simulink model "StarshipSystemModel"  (R2025b)
settings: Solver=VariableStepAuto  StartTime=0.0  StopTime=10.0  RelTol=1e-3
model workspace (MAT data in the model file):
  ActiveGNCMode : Simulink.Bus (value not decoded)
  AerodynamicControlCommand : Simulink.Bus (value not decoded)
  AerodynamicLoad : Simulink.Bus (value not decoded)
  AggregatedStream : Simulink.Bus (value not decoded)
  AllocatedEffectorDemand : Simulink.Bus (value not decoded)
  AttitudeControlDemand : Simulink.Bus (value not decoded)
  AttitudeGuidanceCommand : Simulink.Bus (value not decoded)
  AttitudeRateState : Simulink.Bus (value not decoded)
  AutogenousPressurantGas : Simulink.ConnectionBus (value not decoded)
  CandidateFaultIndication : Simulink.Bus (value not decoded)
  CombustionGasFeed : Simulink.ConnectionBus (value not decoded)
  CommandPathHealth : Simulink.Bus (value not decoded)
  ControlMode : Simulink.ValueType (value not decoded)
  DownlinkSignal : Simulink.Bus (value not decoded)
  ElectricalPower : Simulink.ConnectionBus (value not decoded)
  EngineTelemetry : Simulink.Bus (value not decoded)
  ExecutionContext : Simulink.Bus (value not decoded)
  FaultDiagnosisResult : Simulink.Bus (value not decoded)
  GNCDataContext : Simulink.Bus (value not decoded)
  GNCHealthState : Simulink.Bus (value not decoded)
  GNCStateEstimate : Simulink.Bus (value not decoded)
  GimbalAngle : Simulink.ValueType (value not decoded)
  GimbalMotion : Simulink.ConnectionBus (value not decoded)
  GroundCheckoutLink : Simulink.Bus (value not decoded)
  GroundPressurantSupply : Simulink.ConnectionBus (value not decoded)
  GuidanceConstraints : Simulink.Bus (value not decoded)
  GuidanceMode : Simulink.ValueType (value not decoded)
  LinkHealth : Simulink.Bus (value not decoded)
  LiquidPropellantFeed : Simulink.ConnectionBus (value not decoded)
  MechanicalMotion : Simulink.ConnectionBus (value not decoded)
  MechanismPosition : Simulink.Bus (value not decoded)
  ModeTransitionContext : Simulink.Bus (value not decoded)
  NavigationAidingData : Simulink.Bus (value not decoded)
  NavigationEstimate : Simulink.Bus (value not decoded)
  NavigationHealthStatus : Simulink.Bus (value not decoded)
  NavigationMeasurementSet : Simulink.Bus (value not decoded)
  PercentThrottle : Simulink.ValueType (value not decoded)
  PneumaticActuationGas : Simulink.ConnectionBus (value not decoded)
  PowerConversionStatus : Simulink.Bus (value not decoded)
  PowerDistributionStatus : Simulink.Bus (value not decoded)
  PowerHealthStatus : Simulink.Bus (value not decoded)
  PowerManagementCommand : Simulink.Bus (value not decoded)
  PowerStorageStatus : Simulink.Bus (value not decoded)
  ProtectedThermalState : Simulink.Bus (value not decoded)
  ProtectionIsolationStatus : Simulink.Bus (value not decoded)
  PurgeGasSupply : Simulink.ConnectionBus (value not decoded)
  RCSPulseCommand : Simulink.Bus (value not decoded)
  RCSTelemetry : Simulink.Bus (value not decoded)
  RFFeed : Simulink.ConnectionBus (value not decoded)
  RecoveryMechanismCommand : Simulink.Bus (value not decoded)
  RollThrottleBias : Simulink.ValueType (value not decoded)
  SafetyOverride : Simulink.ValueType (value not decoded)
  SafetyStateStatus : Simulink.Bus (value not decoded)
  ShapedControlDemand : Simulink.Bus (value not decoded)
  SpinStartIgniterGas : Simulink.ConnectionBus (value not decoded)
  StageMechanicalBoundary : Simulink.ConnectionBus (value not decoded)
  StructuralLoad : Simulink.ConnectionBus (value not decoded)
  StructureHealthStatus : Simulink.Bus (value not decoded)
  SubsystemHealthEvidence : Simulink.Bus (value not decoded)
  SubsystemStatusTelemetry : Simulink.Bus (value not decoded)
  TankTelemetry : Simulink.Bus (value not decoded)
  ThermalMonitoringCommand : Simulink.Bus (value not decoded)
  ThermalNetwork : Simulink.ConnectionBus (value not decoded)
  ThrustLoad : Simulink.ConnectionBus (value not decoded)
  TrajectoryGuidanceCommand : Simulink.Bus (value not decoded)
  TrajectoryReference : Simulink.Bus (value not decoded)
  TranslationalControlDemand : Simulink.Bus (value not decoded)
  TranslationalState : Simulink.Bus (value not decoded)
  UplinkSignal : Simulink.Bus (value not decoded)
  ValidatedControlDemand : Simulink.Bus (value not decoded)
  ValveCommand : Simulink.ValueType (value not decoded)
  VehicleStructureState : Simulink.Bus (value not decoded)
  VerifiedCommand : Simulink.Bus (value not decoded)
  VideoStream : Simulink.Bus (value not decoded)
undefined symbols (not defined in the file): ACR, ACT, ASM, ATM, BCR, BDQ, BDR, BDX, BEC, BFC, BHV, BIP, BLM, BNZ, BPI, BPR, BPV, BRX, BSM, BTA, BTP, BVC, BVE, BVV, CAA, CAM, CAS, CAT, CLM, COM, CRS, CTL, CTR, DAQ, ESC, EXT, FCR, FDB, FDE, FEX, FHI, FHM, FIC, FIS, FMG, FSC, GAP, GCM, GMD, GNC, GND, GPH, GTR, HDN, HIA, HSI, IF, INT, LOC, NAI ... (+45)
(part 3 of 8)

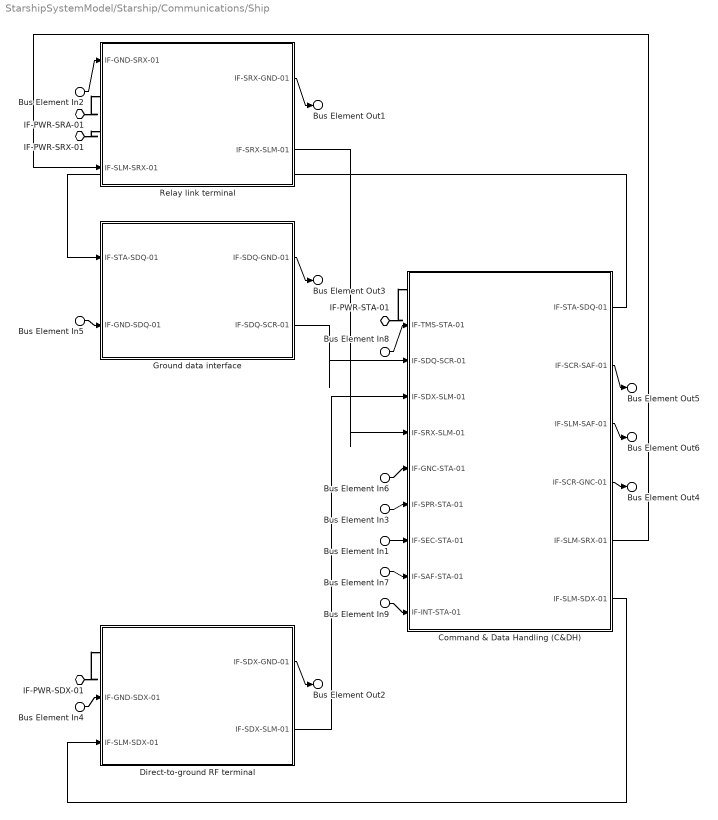
== system StarshipSystemModel/Starship/Communications/Ship ==
  Bus Element In8 : Inport  PortName=IF-TMS-STA-01
  Bus Element In6 : Inport  Port=2  PortName=IF-GNC-STA-01
  Bus Element In3 : Inport  Port=3  PortName=IF-SPR-STA-01
  Bus Element In1 : Inport  Port=4  PortName=IF-SEC-STA-01
  Bus Element In2 : Inport  Port=5  PortName=IF-GND-SRX-01
  Bus Element In4 : Inport  Port=6  PortName=IF-GND-SDX-01
  Bus Element In5 : Inport  Port=7  PortName=IF-GND-SDQ-01
  Bus Element In7 : Inport  Port=8  PortName=IF-SAF-STA-01
  Bus Element In9 : Inport  Port=9  PortName=IF-INT-STA-01
  Command & Data Handling (C&DH) : Subsystem
      settings: PortSchema="{\"entries\":[{\"content\":{\"headerSize\":26,\"margin\":15,\"minimumSpacing\":25,\"sides\":[{\"content\":{\"connectorIds\":[\"LConn1\",\"In1\",\"In2\",\"In3\",\"In4\",\"In5\",\"In6\",\"In7\",\"In8\",\"In9\"]},\"type\":\"ConnectorPlacement.EquallySpacedRectSide\",\"uuid\":\"57d8a002-ec9a-4125-b797-7e7c6712bf02\"},{\"content\":{\"connectorIds\":[\"Out1\",\"Out2\",\"Out3\",\"Out4\",\"Out5\",\"Out6\"],\"side\":\"RIGHT\"},\"type\":\"ConnectorPlacement.EquallySpacedRectSide\",\"uuid\":\"9c166a96-12fc-4382-8ebe-da88da7fda26\"},{\"content\":{\"side\":\"TOP\"},\"type\":\"ConnectorPlacement.EquallySpacedRectSide\",\"uuid\":\"d709cb41-f5aa-4a2a-ad2b-35894222a9c1\"}]},\"type\":\"ConnectorPlacement.EquallySpacedConnector\",\"uuid\":\"04bb3772-118b-42d1-ac15-43c1b901053a\"}],\"packageUris\":[\"http://schema.mathworks.com/mf0/Connector/R2020b\"],\"version\":\"1.0\"}"
  Direct-to-ground RF terminal : Subsystem
      settings: PortSchema="{\"entries\":[{\"content\":{\"headerSize\":26,\"margin\":15,\"minimumSpacing\":25,\"sides\":[{\"content\":{\"connectorIds\":[\"LConn1\",\"In1\",\"In2\"]},\"type\":\"ConnectorPlacement.EquallySpacedRectSide\",\"uuid\":\"57d8a002-ec9a-4125-b797-7e7c6712bf02\"},{\"content\":{\"connectorIds\":[\"Out1\",\"Out2\"],\"side\":\"RIGHT\"},\"type\":\"ConnectorPlacement.EquallySpacedRectSide\",\"uuid\":\"9c166a96-12fc-4382-8ebe-da88da7fda26\"},{\"content\":{\"side\":\"TOP\"},\"type\":\"ConnectorPlacement.EquallySpacedRectSide\",\"uuid\":\"d709cb41-f5aa-4a2a-ad2b-35894222a9c1\"}]},\"type\":\"ConnectorPlacement.EquallySpacedConnector\",\"uuid\":\"04bb3772-118b-42d1-ac15-43c1b901053a\"}],\"packageUris\":[\"http://schema.mathworks.com/mf0/Connector/R2020b\"],\"version\":\"1.0\"}"
  Ground data interface : Subsystem
      settings: PortSchema="{\"entries\":[{\"content\":{\"headerSize\":26,\"margin\":15,\"minimumSpacing\":25,\"sides\":[{\"content\":{\"connectorIds\":[\"In1\",\"In2\"]},\"type\":\"ConnectorPlacement.EquallySpacedRectSide\",\"uuid\":\"57d8a002-ec9a-4125-b797-7e7c6712bf02\"},{\"content\":{\"connectorIds\":[\"Out1\",\"Out2\"],\"side\":\"RIGHT\"},\"type\":\"ConnectorPlacement.EquallySpacedRectSide\",\"uuid\":\"9c166a96-12fc-4382-8ebe-da88da7fda26\"},{\"content\":{\"side\":\"TOP\"},\"type\":\"ConnectorPlacement.EquallySpacedRectSide\",\"uuid\":\"d709cb41-f5aa-4a2a-ad2b-35894222a9c1\"}]},\"type\":\"ConnectorPlacement.EquallySpacedConnector\",\"uuid\":\"04bb3772-118b-42d1-ac15-43c1b901053a\"}],\"packageUris\":[\"http://schema.mathworks.com/mf0/Connector/R2020b\"],\"version\":\"1.0\"}"
  Relay link terminal : Subsystem
      settings: PortSchema="{\"entries\":[{\"content\":{\"headerSize\":26,\"margin\":15,\"minimumSpacing\":25,\"sides\":[{\"content\":{\"connectorIds\":[\"In1\",\"LConn1\",\"LConn2\",\"In2\"]},\"type\":\"ConnectorPlacement.EquallySpacedRectSide\",\"uuid\":\"57d8a002-ec9a-4125-b797-7e7c6712bf02\"},{\"content\":{\"connectorIds\":[\"Out1\",\"Out2\"],\"side\":\"RIGHT\"},\"type\":\"ConnectorPlacement.EquallySpacedRectSide\",\"uuid\":\"9c166a96-12fc-4382-8ebe-da88da7fda26\"},{\"content\":{\"side\":\"TOP\"},\"type\":\"ConnectorPlacement.EquallySpacedRectSide\",\"uuid\":\"d709cb41-f5aa-4a2a-ad2b-35894222a9c1\"}]},\"type\":\"ConnectorPlacement.EquallySpacedConnector\",\"uuid\":\"04bb3772-118b-42d1-ac15-43c1b901053a\"}],\"packageUris\":[\"http://schema.mathworks.com/mf0/Connector/R2020b\"],\"version\":\"1.0\"}"
  IF-PWR-SRA-01 : PMIOPort  Side=Left  ConnectionType=Bus: ElectricalPower
  IF-PWR-SRX-01 : PMIOPort  Port=2  Side=Left  ConnectionType=Bus: ElectricalPower
  IF-PWR-SDX-01 : PMIOPort  Port=3  Side=Left  ConnectionType=Bus: ElectricalPower
  IF-PWR-STA-01 : PMIOPort  Port=4  Side=Left  ConnectionType=Bus: ElectricalPower
  Bus Element Out2 : Outport  PortName=IF-SDX-GND-01
  Bus Element Out1 : Outport  Port=2  PortName=IF-SRX-GND-01
  Bus Element Out3 : Outport  Port=3  PortName=IF-SDQ-GND-01
  Bus Element Out4 : Outport  Port=4  PortName=IF-SCR-GNC-01
  Bus Element Out5 : Outport  Port=5  PortName=IF-SCR-SAF-01
  Bus Element Out6 : Outport  Port=6  PortName=IF-SLM-SAF-01
  wires:
  Relay link terminal/2(IF-SRX-SLM-01) -> Command & Data Handling (C&DH)/4(IF-SRX-SLM-01)
  Bus Element In1/1 -> Command & Data Handling (C&DH)/7(IF-SEC-STA-01)
  Relay link terminal/1(IF-SRX-GND-01) -> Bus Element Out1/1
  Bus Element In2/1 -> Relay link terminal/1(IF-GND-SRX-01)
  Command & Data Handling (C&DH)/4(IF-SCR-GNC-01) -> Bus Element Out4/1
  Bus Element In5/1 -> Ground data interface/2(IF-GND-SDQ-01)
  Command & Data Handling (C&DH)/2(IF-SCR-SAF-01) -> Bus Element Out5/1
  Bus Element In4/1 -> Direct-to-ground RF terminal/1(IF-GND-SDX-01)
  Ground data interface/1(IF-SDQ-GND-01) -> Bus Element Out3/1
  Ground data interface/2(IF-SDQ-SCR-01) -> Command & Data Handling (C&DH)/2(IF-SDQ-SCR-01)
  Bus Element In6/1 -> Command & Data Handling (C&DH)/5(IF-GNC-STA-01)
  Bus Element In3/1 -> Command & Data Handling (C&DH)/6(IF-SPR-STA-01)
  Command & Data Handling (C&DH)/6(IF-SLM-SDX-01) -> Direct-to-ground RF terminal/2(IF-SLM-SDX-01)
  Bus Element In7/1 -> Command & Data Handling (C&DH)/8(IF-SAF-STA-01)
  Direct-to-ground RF terminal/1(IF-SDX-GND-01) -> Bus Element Out2/1
  Direct-to-ground RF terminal/2(IF-SDX-SLM-01) -> Command & Data Handling (C&DH)/3(IF-SDX-SLM-01)
  Command & Data Handling (C&DH)/1(IF-STA-SDQ-01) -> Ground data interface/1(IF-STA-SDQ-01)
  Command & Data Handling (C&DH)/3(IF-SLM-SAF-01) -> Bus Element Out6/1
  Command & Data Handling (C&DH)/5(IF-SLM-SRX-01) -> Relay link terminal/2(IF-SLM-SRX-01)
  Bus Element In8/1 -> Command & Data Handling (C&DH)/1(IF-TMS-STA-01)
  Bus Element In9/1 -> Command & Data Handling (C&DH)/9(IF-INT-STA-01)
  connections:
  IF-PWR-SRA-01/RConn1 -- Relay link terminal/LConn1
  IF-PWR-SRX-01/RConn1 -- Relay link terminal/LConn2
  IF-PWR-SDX-01/RConn1 -- Direct-to-ground RF terminal/LConn1
  IF-PWR-STA-01/RConn1 -- Command & Data Handling (C&DH)/LConn1

== system StarshipSystemModel/Starship/GNC/Control Command & Allocation ==
  Bus Element In1 : Inport  PortName=IF-CLM-CAS-01
  Actuator / Subsystem Command Routing : Subsystem
      settings: PortSchema="{\"entries\":[{\"content\":{\"headerSize\":26,\"margin\":15,\"minimumSpacing\":25,\"sides\":[{\"content\":{\"connectorIds\":[\"In1\",\"LConn1\"]},\"type\":\"ConnectorPlacement.EquallySpacedRectSide\",\"uuid\":\"bfc9b5ca-65d3-4883-965c-09cadc06ae86\"},{\"content\":{\"connectorIds\":[\"Out1\",\"Out2\",\"Out3\",\"Out4\",\"Out5\",\"Out6\",\"Out7\",\"Out8\",\"Out9\",\"Out10\"],\"side\":\"RIGHT\"},\"type\":\"ConnectorPlacement.EquallySpacedRectSide\",\"uuid\":\"302eddba-73e5-4bab-ba05-7a4cd66d036f\"},{\"content\":{\"side\":\"TOP\"},\"type\":\"ConnectorPlacement.EquallySpacedRectSide\",\"uuid\":\"ad98d540-1dfa-45ea-9ded-5f35e32eb634\"}]},\"type\":\"ConnectorPlacement.EquallySpacedConnector\",\"uuid\":\"1bda90bf-7ec8-4676-b4c1-6df6810f307f\"}],\"packageUris\":[\"http://schema.mathworks.com/mf0/Connector/R2020b\"],\"version\":\"1.0\"}"
  Command Shaping & Limiting : Subsystem
      settings: PortSchema="{\"entries\":[{\"content\":{\"headerSize\":26,\"margin\":15,\"minimumSpacing\":25,\"sides\":[{\"content\":{\"connectorIds\":[\"In1\"]},\"type\":\"ConnectorPlacement.EquallySpacedRectSide\",\"uuid\":\"bfc9b5ca-65d3-4883-965c-09cadc06ae86\"},{\"content\":{\"connectorIds\":[\"Out1\"],\"side\":\"RIGHT\"},\"type\":\"ConnectorPlacement.EquallySpacedRectSide\",\"uuid\":\"302eddba-73e5-4bab-ba05-7a4cd66d036f\"},{\"content\":{\"side\":\"TOP\"},\"type\":\"ConnectorPlacement.EquallySpacedRectSide\",\"uuid\":\"ad98d540-1dfa-45ea-9ded-5f35e32eb634\"}]},\"type\":\"ConnectorPlacement.EquallySpacedConnector\",\"uuid\":\"1bda90bf-7ec8-4676-b4c1-6df6810f307f\"}],\"packageUris\":[\"http://schema.mathworks.com/mf0/Connector/R2020b\"],\"version\":\"1.0\"}"
  Control Allocation : Subsystem
      settings: PortSchema="{\"entries\":[{\"content\":{\"headerSize\":26,\"margin\":15,\"minimumSpacing\":25,\"sides\":[{\"content\":{\"connectorIds\":[\"In1\"]},\"type\":\"ConnectorPlacement.EquallySpacedRectSide\",\"uuid\":\"bfc9b5ca-65d3-4883-965c-09cadc06ae86\"},{\"content\":{\"connectorIds\":[\"Out1\"],\"side\":\"RIGHT\"},\"type\":\"ConnectorPlacement.EquallySpacedRectSide\",\"uuid\":\"302eddba-73e5-4bab-ba05-7a4cd66d036f\"},{\"content\":{\"side\":\"TOP\"},\"type\":\"ConnectorPlacement.EquallySpacedRectSide\",\"uuid\":\"ad98d540-1dfa-45ea-9ded-5f35e32eb634\"}]},\"type\":\"ConnectorPlacement.EquallySpacedConnector\",\"uuid\":\"1bda90bf-7ec8-4676-b4c1-6df6810f307f\"}],\"packageUris\":[\"http://schema.mathworks.com/mf0/Connector/R2020b\"],\"version\":\"1.0\"}"
  IF-PWR-GNC-01 : PMIOPort  Side=Left  ConnectionType=Bus: ElectricalPower
  Bus Element Out9 : Outport  PortName=IF-GNC-SPR-01
  Bus Element Out8 : Outport  Port=2  PortName=IF-GNC-BPR-01
  Bus Element Out7 : Outport  Port=3  PortName=IF-GNC-SFC-01
  Bus Element Out6 : Outport  Port=4  PortName=IF-GNC-BFC-01
  Bus Element Out5 : Outport  Port=5  PortName=IF-GNC-RCT-01
  Bus Element Out4 : Outport  Port=6  PortName=IF-GNC-TVC-01
  Bus Element Out3 : Outport  Port=7  PortName=IF-GNC-SEC-01
  Bus Element Out2 : Outport  Port=8  PortName=IF-GNC-BEC-01
  Bus Element Out1 : Outport  Port=9  PortName=IF-CRS-FHM-01
  Bus Element Out10 : Outport  Port=10  PortName=IF-GNC-ACT-01
  wires:
  Actuator / Subsystem Command Routing/4(IF-GNC-BFC-01) -> Bus Element Out6/1
  Actuator / Subsystem Command Routing/2(IF-GNC-BPR-01) -> Bus Element Out8/1
  Command Shaping & Limiting/1(IF-CAS-CAA-01) -> Control Allocation/1(IF-CAS-CAA-01)
  Bus Element In1/1 -> Command Shaping & Limiting/1(IF-CLM-CAS-01)
  Actuator / Subsystem Command Routing/5(IF-GNC-RCT-01) -> Bus Element Out5/1
  Actuator / Subsystem Command Routing/3(IF-GNC-SFC-01) -> Bus Element Out7/1
  Actuator / Subsystem Command Routing/1(IF-GNC-SPR-01) -> Bus Element Out9/1
  Actuator / Subsystem Command Routing/7(IF-GNC-SEC-01) -> Bus Element Out3/1
  Control Allocation/1(IF-CAA-CRS-01) -> Actuator / Subsystem Command Routing/1(IF-CAA-CRS-01)
  Actuator / Subsystem Command Routing/6(IF-GNC-TVC-01) -> Bus Element Out4/1
  Actuator / Subsystem Command Routing/8(IF-GNC-BEC-01) -> Bus Element Out2/1
  Actuator / Subsystem Command Routing/9(IF-CRS-FHM-01) -> Bus Element Out1/1
  Actuator / Subsystem Command Routing/10(IF-GNC-ACT-01) -> Bus Element Out10/1
  connections:
  IF-PWR-GNC-01/RConn1 -- Actuator / Subsystem Command Routing/LConn1

== system StarshipSystemModel/Starship/GNC/Flight Control ==
  Bus Element In3 : Inport  PortName=IF-GPH-CAT-01
  Bus Element In4 : Inport  Port=2  PortName=IF-GPH-CTR-01
  Bus Element In2 : Inport  Port=3  PortName=IF-NSE-CTR-01
  Bus Element In1 : Inport  Port=4  PortName=IF-NSE-CAT-01
  Bus Element In5 : Inport  Port=5  PortName=IF-FMG-CAM-01
  Attitude / Rate Control : Subsystem
      settings: PortSchema="{\"entries\":[{\"content\":{\"headerSize\":26,\"margin\":15,\"minimumSpacing\":25,\"sides\":[{\"content\":{\"connectorIds\":[\"In1\",\"In2\",\"In3\"]},\"type\":\"ConnectorPlacement.EquallySpacedRectSide\",\"uuid\":\"bfc9b5ca-65d3-4883-965c-09cadc06ae86\"},{\"content\":{\"connectorIds\":[\"Out1\"],\"side\":\"RIGHT\"},\"type\":\"ConnectorPlacement.EquallySpacedRectSide\",\"uuid\":\"302eddba-73e5-4bab-ba05-7a4cd66d036f\"},{\"content\":{\"side\":\"TOP\"},\"type\":\"ConnectorPlacement.EquallySpacedRectSide\",\"uuid\":\"ad98d540-1dfa-45ea-9ded-5f35e32eb634\"}]},\"type\":\"ConnectorPlacement.EquallySpacedConnector\",\"uuid\":\"1bda90bf-7ec8-4676-b4c1-6df6810f307f\"}],\"packageUris\":[\"http://schema.mathworks.com/mf0/Connector/R2020b\"],\"version\":\"1.0\"}"
  Control-Law Monitoring & Limiting : Subsystem
      settings: PortSchema="{\"entries\":[{\"content\":{\"headerSize\":26,\"margin\":15,\"minimumSpacing\":25,\"sides\":[{\"content\":{\"connectorIds\":[\"In1\",\"In2\"]},\"type\":\"ConnectorPlacement.EquallySpacedRectSide\",\"uuid\":\"bfc9b5ca-65d3-4883-965c-09cadc06ae86\"},{\"content\":{\"connectorIds\":[\"Out1\"],\"side\":\"RIGHT\"},\"type\":\"ConnectorPlacement.EquallySpacedRectSide\",\"uuid\":\"302eddba-73e5-4bab-ba05-7a4cd66d036f\"},{\"content\":{\"side\":\"TOP\"},\"type\":\"ConnectorPlacement.EquallySpacedRectSide\",\"uuid\":\"ad98d540-1dfa-45ea-9ded-5f35e32eb634\"}]},\"type\":\"ConnectorPlacement.EquallySpacedConnector\",\"uuid\":\"1bda90bf-7ec8-4676-b4c1-6df6810f307f\"}],\"packageUris\":[\"http://schema.mathworks.com/mf0/Connector/R2020b\"],\"version\":\"1.0\"}"
  Control-Mode Management : Subsystem
      settings: PortSchema="{\"entries\":[{\"content\":{\"headerSize\":26,\"margin\":15,\"minimumSpacing\":25,\"sides\":[{\"content\":{\"connectorIds\":[\"In1\"]},\"type\":\"ConnectorPlacement.EquallySpacedRectSide\",\"uuid\":\"bfc9b5ca-65d3-4883-965c-09cadc06ae86\"},{\"content\":{\"connectorIds\":[\"Out1\",\"Out2\"],\"side\":\"RIGHT\"},\"type\":\"ConnectorPlacement.EquallySpacedRectSide\",\"uuid\":\"302eddba-73e5-4bab-ba05-7a4cd66d036f\"},{\"content\":{\"side\":\"TOP\"},\"type\":\"ConnectorPlacement.EquallySpacedRectSide\",\"uuid\":\"ad98d540-1dfa-45ea-9ded-5f35e32eb634\"}]},\"type\":\"ConnectorPlacement.EquallySpacedConnector\",\"uuid\":\"1bda90bf-7ec8-4676-b4c1-6df6810f307f\"}],\"packageUris\":[\"http://schema.mathworks.com/mf0/Connector/R2020b\"],\"version\":\"1.0\"}"
  Trajectory / Translational Control : Subsystem
      settings: PortSchema="{\"entries\":[{\"content\":{\"headerSize\":26,\"margin\":15,\"minimumSpacing\":25,\"sides\":[{\"content\":{\"connectorIds\":[\"In1\",\"In2\",\"In3\"]},\"type\":\"ConnectorPlacement.EquallySpacedRectSide\",\"uuid\":\"bfc9b5ca-65d3-4883-965c-09cadc06ae86\"},{\"content\":{\"connectorIds\":[\"Out1\"],\"side\":\"RIGHT\"},\"type\":\"ConnectorPlacement.EquallySpacedRectSide\",\"uuid\":\"302eddba-73e5-4bab-ba05-7a4cd66d036f\"},{\"content\":{\"side\":\"TOP\"},\"type\":\"ConnectorPlacement.EquallySpacedRectSide\",\"uuid\":\"ad98d540-1dfa-45ea-9ded-5f35e32eb634\"}]},\"type\":\"ConnectorPlacement.EquallySpacedConnector\",\"uuid\":\"1bda90bf-7ec8-4676-b4c1-6df6810f307f\"}],\"packageUris\":[\"http://schema.mathworks.com/mf0/Connector/R2020b\"],\"version\":\"1.0\"}"
  Bus Element Out1 : Outport  PortName=IF-CLM-CAS-01
  wires:
  Bus Element In1/1 -> Attitude / Rate Control/2(IF-NSE-CAT-01)
  Bus Element In4/1 -> Trajectory / Translational Control/2(IF-GPH-CTR-01)
  Control-Mode Management/1(IF-CAM-CAT-01) -> Attitude / Rate Control/3(IF-CAM-CAT-01)
  Bus Element In3/1 -> Attitude / Rate Control/1(IF-GPH-CAT-01)
  Bus Element In2/1 -> Trajectory / Translational Control/1(IF-NSE-CTR-01)
  Bus Element In5/1 -> Control-Mode Management/1(IF-FMG-CAM-01)
  Control-Mode Management/2(IF-CAM-CTR-01) -> Trajectory / Translational Control/3(IF-CAM-CTR-01)
  Trajectory / Translational Control/1(IF-CTR-CLM-01) -> Control-Law Monitoring & Limiting/1(IF-CTR-CLM-01)
  Attitude / Rate Control/1(IF-CAT-CLM-01) -> Control-Law Monitoring & Limiting/2(IF-CAT-CLM-01)
  Control-Law Monitoring & Limiting/1(IF-CLM-CAS-01) -> Bus Element Out1/1

== system StarshipSystemModel/Starship/GNC/GNC Flight Software & Mode Management ==
  Bus Element In6 : Inport  PortName=IF-SAF-FHM-01
  Bus Element In5 : Inport  Port=2  PortName=IF-SCR-GNC-01
  Bus Element In4 : Inport  Port=3  PortName=IF-BCR-GNC-01
  Bus Element In3 : Inport  Port=4  PortName=IF-TVC-GNC-01
  Bus Element In1 : Inport  Port=5  PortName=IF-NVI-FHM-01
  Bus Element In2 : Inport  Port=6  PortName=IF-CRS-FHM-01
  GNC Data & Interface Management : Subsystem
      settings: PortSchema="{\"entries\":[{\"content\":{\"headerSize\":26,\"margin\":15,\"minimumSpacing\":25,\"sides\":[{\"content\":{\"connectorIds\":[\"In2\",\"In1\",\"In3\"]},\"type\":\"ConnectorPlacement.EquallySpacedRectSide\",\"uuid\":\"bfc9b5ca-65d3-4883-965c-09cadc06ae86\"},{\"content\":{\"connectorIds\":[\"Out1\",\"Out2\",\"Out3\"],\"side\":\"RIGHT\"},\"type\":\"ConnectorPlacement.EquallySpacedRectSide\",\"uuid\":\"302eddba-73e5-4bab-ba05-7a4cd66d036f\"},{\"content\":{\"side\":\"TOP\"},\"type\":\"ConnectorPlacement.EquallySpacedRectSide\",\"uuid\":\"ad98d540-1dfa-45ea-9ded-5f35e32eb634\"},{\"content\":{\"side\":\"BOTTOM\"},\"type\":\"ConnectorPlacement.EquallySpacedRectSide\",\"uuid\":\"ee596e90-1eb5-469d-9fa4-539f9d2bb748\"}]},\"type\":\"ConnectorPlacement.EquallySpacedConnector\",\"uuid\":\"1bda90bf-7ec8-4676-b4c1-6df6810f307f\"}],\"packageUris\":[\"http://schema.mathworks.com/mf0/Connector/R2020b\"],\"version\":\"1.0\"}"
  GNC Function Execution : Subsystem
      settings: PortSchema="{\"entries\":[{\"content\":{\"headerSize\":26,\"margin\":15,\"minimumSpacing\":25,\"sides\":[{\"content\":{\"connectorIds\":[\"In1\"]},\"type\":\"ConnectorPlacement.EquallySpacedRectSide\",\"uuid\":\"bfc9b5ca-65d3-4883-965c-09cadc06ae86\"},{\"content\":{\"connectorIds\":[\"Out1\"],\"side\":\"RIGHT\"},\"type\":\"ConnectorPlacement.EquallySpacedRectSide\",\"uuid\":\"302eddba-73e5-4bab-ba05-7a4cd66d036f\"},{\"content\":{\"side\":\"TOP\"},\"type\":\"ConnectorPlacement.EquallySpacedRectSide\",\"uuid\":\"ad98d540-1dfa-45ea-9ded-5f35e32eb634\"}]},\"type\":\"ConnectorPlacement.EquallySpacedConnector\",\"uuid\":\"1bda90bf-7ec8-4676-b4c1-6df6810f307f\"}],\"packageUris\":[\"http://schema.mathworks.com/mf0/Connector/R2020b\"],\"version\":\"1.0\"}"
  GNC Health Monitoring / Fault Response : Subsystem
      settings: PortSchema="{\"entries\":[{\"content\":{\"headerSize\":26,\"margin\":15,\"minimumSpacing\":25,\"sides\":[{\"content\":{\"connectorIds\":[\"In1\",\"In2\",\"In3\"]},\"type\":\"ConnectorPlacement.EquallySpacedRectSide\",\"uuid\":\"bfc9b5ca-65d3-4883-965c-09cadc06ae86\"},{\"content\":{\"connectorIds\":[\"Out1\",\"Out2\",\"Out3\"],\"side\":\"RIGHT\"},\"type\":\"ConnectorPlacement.EquallySpacedRectSide\",\"uuid\":\"302eddba-73e5-4bab-ba05-7a4cd66d036f\"},{\"content\":{\"side\":\"TOP\"},\"type\":\"ConnectorPlacement.EquallySpacedRectSide\",\"uuid\":\"ad98d540-1dfa-45ea-9ded-5f35e32eb634\"}]},\"type\":\"ConnectorPlacement.EquallySpacedConnector\",\"uuid\":\"1bda90bf-7ec8-4676-b4c1-6df6810f307f\"}],\"packageUris\":[\"http://schema.mathworks.com/mf0/Connector/R2020b\"],\"version\":\"1.0\"}"
  GNC Mode Management : Subsystem
      settings: PortSchema="{\"entries\":[{\"content\":{\"headerSize\":26,\"margin\":15,\"minimumSpacing\":25,\"sides\":[{\"content\":{\"connectorIds\":[\"In1\",\"In2\"]},\"type\":\"ConnectorPlacement.EquallySpacedRectSide\",\"uuid\":\"bfc9b5ca-65d3-4883-965c-09cadc06ae86\"},{\"content\":{\"connectorIds\":[\"Out1\",\"Out2\"],\"side\":\"RIGHT\"},\"type\":\"ConnectorPlacement.EquallySpacedRectSide\",\"uuid\":\"302eddba-73e5-4bab-ba05-7a4cd66d036f\"},{\"content\":{\"side\":\"TOP\"},\"type\":\"ConnectorPlacement.EquallySpacedRectSide\",\"uuid\":\"ad98d540-1dfa-45ea-9ded-5f35e32eb634\"}]},\"type\":\"ConnectorPlacement.EquallySpacedConnector\",\"uuid\":\"1bda90bf-7ec8-4676-b4c1-6df6810f307f\"}],\"packageUris\":[\"http://schema.mathworks.com/mf0/Connector/R2020b\"],\"version\":\"1.0\"}"
  Bus Element Out5 : Outport  PortName=IF-GNC-TMS-01
  Bus Element Out4 : Outport  Port=2  PortName=IF-GNC-STA-01
  Bus Element Out3 : Outport  Port=3  PortName=IF-GNC-BTA-01
  Bus Element Out1 : Outport  Port=4  PortName=IF-FMG-GMD-01
  Bus Element Out2 : Outport  Port=5  PortName=IF-FMG-CAM-01
  Bus Element Out6 : Outport  Port=6  PortName=IF-FHM-SAF-01
  wires:
  GNC Health Monitoring / Fault Response/2(IF-GNC-TMS-01) -> Bus Element Out5/1
  Bus Element In2/1 -> GNC Health Monitoring / Fault Response/3(IF-CRS-FHM-01)
  Bus Element In1/1 -> GNC Health Monitoring / Fault Response/2(IF-NVI-FHM-01)
  GNC Data & Interface Management/3(IF-GNC-STA-01) -> Bus Element Out4/1
  GNC Data & Interface Management/1(IF-FDB-FEX-01) -> GNC Function Execution/1(IF-FDB-FEX-01)
  GNC Health Monitoring / Fault Response/1(IF-FHM-FMG-01) -> GNC Mode Management/2(IF-FHM-FMG-01)
  GNC Function Execution/1(IF-FEX-FMG-01) -> GNC Mode Management/1(IF-FEX-FMG-01)
  GNC Data & Interface Management/2(IF-GNC-BTA-01) -> Bus Element Out3/1
  GNC Mode Management/1(IF-FMG-GMD-01) -> Bus Element Out1/1
  GNC Mode Management/2(IF-FMG-CAM-01) -> Bus Element Out2/1
  Bus Element In5/1 -> GNC Data & Interface Management/2(IF-SCR-GNC-01)
  Bus Element In4/1 -> GNC Data & Interface Management/1(IF-BCR-GNC-01)
  Bus Element In3/1 -> GNC Data & Interface Management/3(IF-TVC-GNC-01)
  GNC Health Monitoring / Fault Response/3(IF-FHM-SAF-01) -> Bus Element Out6/1
  Bus Element In6/1 -> GNC Health Monitoring / Fault Response/1(IF-SAF-FHM-01)

== system StarshipSystemModel/Starship/GNC/Guidance & Trajectory Management ==
  Bus Element In1 : Inport  PortName=IF-NSE-GPH-01
  Bus Element In2 : Inport  Port=2  PortName=IF-FMG-GMD-01
  Flight-Phase Guidance : Subsystem
      settings: PortSchema="{\"entries\":[{\"content\":{\"headerSize\":26,\"margin\":15,\"minimumSpacing\":25,\"sides\":[{\"content\":{\"connectorIds\":[\"In1\",\"In2\",\"In3\",\"In4\"]},\"type\":\"ConnectorPlacement.EquallySpacedRectSide\",\"uuid\":\"bfc9b5ca-65d3-4883-965c-09cadc06ae86\"},{\"content\":{\"connectorIds\":[\"Out1\",\"Out2\"],\"side\":\"RIGHT\"},\"type\":\"ConnectorPlacement.EquallySpacedRectSide\",\"uuid\":\"302eddba-73e5-4bab-ba05-7a4cd66d036f\"},{\"content\":{\"side\":\"TOP\"},\"type\":\"ConnectorPlacement.EquallySpacedRectSide\",\"uuid\":\"ad98d540-1dfa-45ea-9ded-5f35e32eb634\"}]},\"type\":\"ConnectorPlacement.EquallySpacedConnector\",\"uuid\":\"1bda90bf-7ec8-4676-b4c1-6df6810f307f\"}],\"packageUris\":[\"http://schema.mathworks.com/mf0/Connector/R2020b\"],\"version\":\"1.0\"}"
  Guidance Constraints & Targeting : Subsystem
      settings: PortSchema="{\"entries\":[{\"content\":{\"headerSize\":26,\"margin\":15,\"minimumSpacing\":25,\"sides\":[{\"content\":{},\"type\":\"ConnectorPlacement.EquallySpacedRectSide\",\"uuid\":\"bfc9b5ca-65d3-4883-965c-09cadc06ae86\"},{\"content\":{\"connectorIds\":[\"Out1\"],\"side\":\"RIGHT\"},\"type\":\"ConnectorPlacement.EquallySpacedRectSide\",\"uuid\":\"302eddba-73e5-4bab-ba05-7a4cd66d036f\"},{\"content\":{\"side\":\"TOP\"},\"type\":\"ConnectorPlacement.EquallySpacedRectSide\",\"uuid\":\"ad98d540-1dfa-45ea-9ded-5f35e32eb634\"}]},\"type\":\"ConnectorPlacement.EquallySpacedConnector\",\"uuid\":\"1bda90bf-7ec8-4676-b4c1-6df6810f307f\"}],\"packageUris\":[\"http://schema.mathworks.com/mf0/Connector/R2020b\"],\"version\":\"1.0\"}"
  Guidance Mode / Transition Logic : Subsystem
      settings: PortSchema="{\"entries\":[{\"content\":{\"headerSize\":26,\"margin\":15,\"minimumSpacing\":25,\"sides\":[{\"content\":{\"connectorIds\":[\"In1\"]},\"type\":\"ConnectorPlacement.EquallySpacedRectSide\",\"uuid\":\"bfc9b5ca-65d3-4883-965c-09cadc06ae86\"},{\"content\":{\"connectorIds\":[\"Out1\"],\"side\":\"RIGHT\"},\"type\":\"ConnectorPlacement.EquallySpacedRectSide\",\"uuid\":\"302eddba-73e5-4bab-ba05-7a4cd66d036f\"},{\"content\":{\"side\":\"TOP\"},\"type\":\"ConnectorPlacement.EquallySpacedRectSide\",\"uuid\":\"ad98d540-1dfa-45ea-9ded-5f35e32eb634\"}]},\"type\":\"ConnectorPlacement.EquallySpacedConnector\",\"uuid\":\"1bda90bf-7ec8-4676-b4c1-6df6810f307f\"}],\"packageUris\":[\"http://schema.mathworks.com/mf0/Connector/R2020b\"],\"version\":\"1.0\"}"
  Trajectory / Reference Management : Subsystem
      settings: PortSchema="{\"entries\":[{\"content\":{\"headerSize\":26,\"margin\":15,\"minimumSpacing\":25,\"sides\":[{\"content\":{},\"type\":\"ConnectorPlacement.EquallySpacedRectSide\",\"uuid\":\"bfc9b5ca-65d3-4883-965c-09cadc06ae86\"},{\"content\":{\"connectorIds\":[\"Out1\"],\"side\":\"RIGHT\"},\"type\":\"ConnectorPlacement.EquallySpacedRectSide\",\"uuid\":\"302eddba-73e5-4bab-ba05-7a4cd66d036f\"},{\"content\":{\"side\":\"TOP\"},\"type\":\"ConnectorPlacement.EquallySpacedRectSide\",\"uuid\":\"ad98d540-1dfa-45ea-9ded-5f35e32eb634\"}]},\"type\":\"ConnectorPlacement.EquallySpacedConnector\",\"uuid\":\"1bda90bf-7ec8-4676-b4c1-6df6810f307f\"}],\"packageUris\":[\"http://schema.mathworks.com/mf0/Connector/R2020b\"],\"version\":\"1.0\"}"
  Bus Element Out1 : Outport  PortName=IF-GPH-CAT-01
  Bus Element Out2 : Outport  Port=2  PortName=IF-GPH-CTR-01
  wires:
  Flight-Phase Guidance/1(IF-GPH-CAT-01) -> Bus Element Out1/1
  Bus Element In1/1 -> Flight-Phase Guidance/1(IF-NSE-GPH-01)
  Bus Element In2/1 -> Guidance Mode / Transition Logic/1(IF-FMG-GMD-01)
  Guidance Mode / Transition Logic/1(IF-GMD-GPH-01) -> Flight-Phase Guidance/4(IF-GMD-GPH-01)
  Trajectory / Reference Management/1(IF-GTR-GPH-01) -> Flight-Phase Guidance/2(IF-GTR-GPH-01)
  Flight-Phase Guidance/2(IF-GPH-CTR-01) -> Bus Element Out2/1
  Guidance Constraints & Targeting/1(IF-GCM-GPH-01) -> Flight-Phase Guidance/3(IF-GCM-GPH-01)

== system StarshipSystemModel/Starship/GNC/Navigation & State Estimation ==
  Bus Element In2 : Inport  PortName=IF-POS-GNC-01
  Bus Element In1 : Inport  Port=2  PortName=IF-TMS-GNC-01
  Measurement Processing : Subsystem
      settings: PortSchema="{\"entries\":[{\"content\":{\"headerSize\":26,\"margin\":15,\"minimumSpacing\":25,\"sides\":[{\"content\":{\"connectorIds\":[\"In1\"]},\"type\":\"ConnectorPlacement.EquallySpacedRectSide\",\"uuid\":\"bfc9b5ca-65d3-4883-965c-09cadc06ae86\"},{\"content\":{\"connectorIds\":[\"Out1\"],\"side\":\"RIGHT\"},\"type\":\"ConnectorPlacement.EquallySpacedRectSide\",\"uuid\":\"302eddba-73e5-4bab-ba05-7a4cd66d036f\"},{\"content\":{\"side\":\"TOP\"},\"type\":\"ConnectorPlacement.EquallySpacedRectSide\",\"uuid\":\"ad98d540-1dfa-45ea-9ded-5f35e32eb634\"}]},\"type\":\"ConnectorPlacement.EquallySpacedConnector\",\"uuid\":\"1bda90bf-7ec8-4676-b4c1-6df6810f307f\"}],\"packageUris\":[\"http://schema.mathworks.com/mf0/Connector/R2020b\"],\"version\":\"1.0\"}"
  Navigation Aiding Integration : Subsystem
      settings: PortSchema="{\"entries\":[{\"content\":{\"headerSize\":26,\"margin\":15,\"minimumSpacing\":25,\"sides\":[{\"content\":{},\"type\":\"ConnectorPlacement.EquallySpacedRectSide\",\"uuid\":\"bfc9b5ca-65d3-4883-965c-09cadc06ae86\"},{\"content\":{\"connectorIds\":[\"Out1\"],\"side\":\"RIGHT\"},\"type\":\"ConnectorPlacement.EquallySpacedRectSide\",\"uuid\":\"302eddba-73e5-4bab-ba05-7a4cd66d036f\"},{\"content\":{\"side\":\"TOP\"},\"type\":\"ConnectorPlacement.EquallySpacedRectSide\",\"uuid\":\"ad98d540-1dfa-45ea-9ded-5f35e32eb634\"}]},\"type\":\"ConnectorPlacement.EquallySpacedConnector\",\"uuid\":\"1bda90bf-7ec8-4676-b4c1-6df6810f307f\"}],\"packageUris\":[\"http://schema.mathworks.com/mf0/Connector/R2020b\"],\"version\":\"1.0\"}"
  Navigation Validity & Integrity : Subsystem
      settings: PortSchema="{\"entries\":[{\"content\":{\"headerSize\":26,\"margin\":15,\"minimumSpacing\":25,\"sides\":[{\"content\":{\"connectorIds\":[\"In1\"]},\"type\":\"ConnectorPlacement.EquallySpacedRectSide\",\"uuid\":\"bfc9b5ca-65d3-4883-965c-09cadc06ae86\"},{\"content\":{\"connectorIds\":[\"Out1\"],\"side\":\"RIGHT\"},\"type\":\"ConnectorPlacement.EquallySpacedRectSide\",\"uuid\":\"302eddba-73e5-4bab-ba05-7a4cd66d036f\"},{\"content\":{\"side\":\"TOP\"},\"type\":\"ConnectorPlacement.EquallySpacedRectSide\",\"uuid\":\"ad98d540-1dfa-45ea-9ded-5f35e32eb634\"}]},\"type\":\"ConnectorPlacement.EquallySpacedConnector\",\"uuid\":\"1bda90bf-7ec8-4676-b4c1-6df6810f307f\"}],\"packageUris\":[\"http://schema.mathworks.com/mf0/Connector/R2020b\"],\"version\":\"1.0\"}"
  State Estimation : Subsystem
      settings: PortSchema="{\"entries\":[{\"content\":{\"headerSize\":26,\"margin\":15,\"minimumSpacing\":25,\"sides\":[{\"content\":{\"connectorIds\":[\"In1\",\"In2\",\"In3\"]},\"type\":\"ConnectorPlacement.EquallySpacedRectSide\",\"uuid\":\"bfc9b5ca-65d3-4883-965c-09cadc06ae86\"},{\"content\":{\"connectorIds\":[\"Out1\",\"Out2\",\"Out3\",\"Out4\"],\"side\":\"RIGHT\"},\"type\":\"ConnectorPlacement.EquallySpacedRectSide\",\"uuid\":\"302eddba-73e5-4bab-ba05-7a4cd66d036f\"},{\"content\":{\"side\":\"TOP\"},\"type\":\"ConnectorPlacement.EquallySpacedRectSide\",\"uuid\":\"ad98d540-1dfa-45ea-9ded-5f35e32eb634\"}]},\"type\":\"ConnectorPlacement.EquallySpacedConnector\",\"uuid\":\"1bda90bf-7ec8-4676-b4c1-6df6810f307f\"}],\"packageUris\":[\"http://schema.mathworks.com/mf0/Connector/R2020b\"],\"version\":\"1.0\"}"
  Bus Element Out1 : Outport  PortName=IF-NSE-GPH-01
  Bus Element Out3 : Outport  Port=2  PortName=IF-NSE-CTR-01
  Bus Element Out2 : Outport  Port=3  PortName=IF-NSE-CAT-01
  Bus Element Out4 : Outport  Port=4  PortName=IF-NVI-FHM-01
  wires:
  Navigation Validity & Integrity/1(IF-NVI-FHM-01) -> Bus Element Out4/1
  State Estimation/3(IF-NSE-CAT-01) -> Bus Element Out2/1
  State Estimation/1(IF-NSE-GPH-01) -> Bus Element Out1/1
  Bus Element In1/1 -> Measurement Processing/1(IF-TMS-GNC-01)
  State Estimation/4(IF-NSE-NVI-01) -> Navigation Validity & Integrity/1(IF-NSE-NVI-01)
  State Estimation/2(IF-NSE-CTR-01) -> Bus Element Out3/1
  Measurement Processing/1(IF-NMP-NSE-01) -> State Estimation/3(IF-NMP-NSE-01)
  Navigation Aiding Integration/1(IF-NAI-NSE-01) -> State Estimation/2(IF-NAI-NSE-01)
  Bus Element In2/1 -> State Estimation/1(IF-POS-GNC-01)

== system StarshipSystemModel/Starship/Power & Electrical Energy/Distributed Energy Storage ==
  Bus Element In1 : Inport  PortName=IF-PMC-BIP-01
  Battery Energy Storage : Subsystem
      settings: PortSchema="{\"entries\":[{\"content\":{\"headerSize\":26,\"margin\":15,\"minimumSpacing\":25,\"sides\":[{\"content\":{},\"type\":\"ConnectorPlacement.EquallySpacedRectSide\",\"uuid\":\"e231466c-79f3-4a10-9258-08b328dbb315\"},{\"content\":{\"connectorIds\":[\"RConn1\"],\"side\":\"RIGHT\"},\"type\":\"ConnectorPlacement.EquallySpacedRectSide\",\"uuid\":\"d7277c0a-5b77-426a-ad5b-7f06851f857a\"},{\"content\":{\"side\":\"TOP\"},\"type\":\"ConnectorPlacement.EquallySpacedRectSide\",\"uuid\":\"72d60576-32e4-4fd9-b552-a617024da2ce\"}]},\"type\":\"ConnectorPlacement.EquallySpacedConnector\",\"uuid\":\"6309e805-37c0-4868-97b0-5f8fd0bed587\"}],\"packageUris\":[\"http://schema.mathworks.com/mf0/Connector/R2020b\"],\"version\":\"1.0\"}"
  Battery Isolation & Protection : Subsystem
      settings: PortSchema="{\"entries\":[{\"content\":{\"headerSize\":26,\"margin\":15,\"minimumSpacing\":25,\"sides\":[{\"content\":{\"connectorIds\":[\"In1\"]},\"type\":\"ConnectorPlacement.EquallySpacedRectSide\",\"uuid\":\"e231466c-79f3-4a10-9258-08b328dbb315\"},{\"content\":{\"connectorIds\":[\"Out1\"],\"side\":\"RIGHT\"},\"type\":\"ConnectorPlacement.EquallySpacedRectSide\",\"uuid\":\"d7277c0a-5b77-426a-ad5b-7f06851f857a\"},{\"content\":{\"side\":\"TOP\"},\"type\":\"ConnectorPlacement.EquallySpacedRectSide\",\"uuid\":\"72d60576-32e4-4fd9-b552-a617024da2ce\"}]},\"type\":\"ConnectorPlacement.EquallySpacedConnector\",\"uuid\":\"6309e805-37c0-4868-97b0-5f8fd0bed587\"}],\"packageUris\":[\"http://schema.mathworks.com/mf0/Connector/R2020b\"],\"version\":\"1.0\"}"
  Battery State Monitoring : Subsystem
      settings: PortSchema="{\"entries\":[{\"content\":{\"headerSize\":26,\"margin\":15,\"minimumSpacing\":25,\"sides\":[{\"content\":{},\"type\":\"ConnectorPlacement.EquallySpacedRectSide\",\"uuid\":\"e231466c-79f3-4a10-9258-08b328dbb315\"},{\"content\":{\"connectorIds\":[\"Out1\"],\"side\":\"RIGHT\"},\"type\":\"ConnectorPlacement.EquallySpacedRectSide\",\"uuid\":\"d7277c0a-5b77-426a-ad5b-7f06851f857a\"},{\"content\":{\"side\":\"TOP\"},\"type\":\"ConnectorPlacement.EquallySpacedRectSide\",\"uuid\":\"72d60576-32e4-4fd9-b552-a617024da2ce\"}]},\"type\":\"ConnectorPlacement.EquallySpacedConnector\",\"uuid\":\"6309e805-37c0-4868-97b0-5f8fd0bed587\"}],\"packageUris\":[\"http://schema.mathworks.com/mf0/Connector/R2020b\"],\"version\":\"1.0\"}"
  IF-BES-INV-01 : PMIOPort  Side=Right  ConnectionType=Bus: ElectricalPower
  Bus Element Out1 : Outport  PortName=IF-BSM-PSM-01
  Bus Element Out2 : Outport  Port=2  PortName=IF-BIP-PIS-01
  wires:
  Bus Element In1/1 -> Battery Isolation & Protection/1(IF-PMC-BIP-01)
  Battery Isolation & Protection/1(IF-BIP-PIS-01) -> Bus Element Out2/1
  Battery State Monitoring/1(IF-BSM-PSM-01) -> Bus Element Out1/1
  connections:
  Battery Energy Storage/RConn1 -- IF-BES-INV-01/RConn1

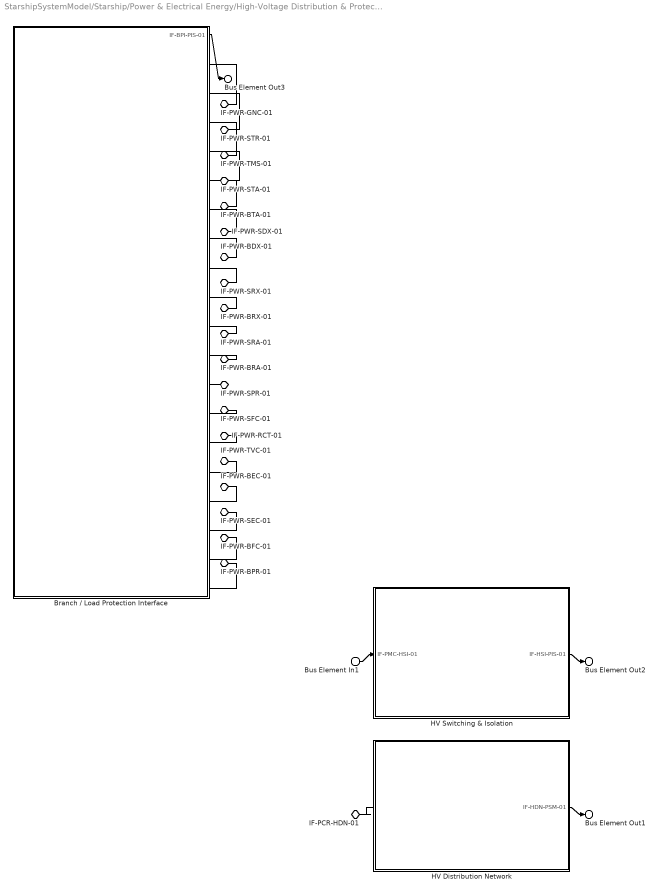
== system StarshipSystemModel/Starship/Power & Electrical Energy/High-Voltage Distribution & Protection ==
  Bus Element In1 : Inport  PortName=IF-PMC-HSI-01
  Branch / Load Protection Interface : Subsystem
      settings: PortSchema="{\"entries\":[{\"content\":{\"headerSize\":26,\"margin\":15,\"minimumSpacing\":25,\"sides\":[{\"content\":{},\"type\":\"ConnectorPlacement.EquallySpacedRectSide\",\"uuid\":\"e231466c-79f3-4a10-9258-08b328dbb315\"},{\"content\":{\"connectorIds\":[\"Out1\",\"RConn1\",\"RConn2\",\"RConn3\",\"RConn4\",\"RConn5\",\"RConn6\",\"RConn7\",\"RConn8\",\"RConn9\",\"RConn10\",\"RConn11\",\"RConn12\",\"RConn13\",\"RConn14\",\"RConn15\",\"RConn16\",\"RConn17\",\"RConn18\",\"RConn19\"],\"side\":\"RIGHT\"},\"type\":\"ConnectorPlacement.EquallySpacedRectSide\",\"uuid\":\"d7277c0a-5b77-426a-ad5b-7f06851f857a\"},{\"content\":{\"side\":\"TOP\"},\"type\":\"ConnectorPlacement.EquallySpacedRectSide\",\"uuid\":\"72d60576-32e4-4fd9-b552-a617024da2ce\"}]},\"type\":\"ConnectorPlacement.EquallySpacedConnector\",\"uuid\":\"6309e805-37c0-4868-97b0-5f8fd0bed587\"}],\"packageUris\":[\"http://schema.mathworks.com/mf0/Connector/R2020b\"],\"version\":\"1.0\"}"
  HV Distribution Network : Subsystem
      settings: PortSchema="{\"entries\":[{\"content\":{\"headerSize\":26,\"margin\":15,\"minimumSpacing\":25,\"sides\":[{\"content\":{\"connectorIds\":[\"LConn1\"]},\"type\":\"ConnectorPlacement.EquallySpacedRectSide\",\"uuid\":\"e231466c-79f3-4a10-9258-08b328dbb315\"},{\"content\":{\"connectorIds\":[\"Out1\"],\"side\":\"RIGHT\"},\"type\":\"ConnectorPlacement.EquallySpacedRectSide\",\"uuid\":\"d7277c0a-5b77-426a-ad5b-7f06851f857a\"},{\"content\":{\"side\":\"TOP\"},\"type\":\"ConnectorPlacement.EquallySpacedRectSide\",\"uuid\":\"72d60576-32e4-4fd9-b552-a617024da2ce\"}]},\"type\":\"ConnectorPlacement.EquallySpacedConnector\",\"uuid\":\"6309e805-37c0-4868-97b0-5f8fd0bed587\"}],\"packageUris\":[\"http://schema.mathworks.com/mf0/Connector/R2020b\"],\"version\":\"1.0\"}"
  HV Switching & Isolation : Subsystem
      settings: PortSchema="{\"entries\":[{\"content\":{\"headerSize\":26,\"margin\":15,\"minimumSpacing\":25,\"sides\":[{\"content\":{\"connectorIds\":[\"In1\"]},\"type\":\"ConnectorPlacement.EquallySpacedRectSide\",\"uuid\":\"e231466c-79f3-4a10-9258-08b328dbb315\"},{\"content\":{\"connectorIds\":[\"Out1\"],\"side\":\"RIGHT\"},\"type\":\"ConnectorPlacement.EquallySpacedRectSide\",\"uuid\":\"d7277c0a-5b77-426a-ad5b-7f06851f857a\"},{\"content\":{\"side\":\"TOP\"},\"type\":\"ConnectorPlacement.EquallySpacedRectSide\",\"uuid\":\"72d60576-32e4-4fd9-b552-a617024da2ce\"}]},\"type\":\"ConnectorPlacement.EquallySpacedConnector\",\"uuid\":\"6309e805-37c0-4868-97b0-5f8fd0bed587\"}],\"packageUris\":[\"http://schema.mathworks.com/mf0/Connector/R2020b\"],\"version\":\"1.0\"}"
  IF-PWR-RCT-01 : PMIOPort  Side=Right  ConnectionType=Bus: ElectricalPower
  IF-PWR-TVC-01 : PMIOPort  Port=2  Side=Right  ConnectionType=Bus: ElectricalPower
  IF-PWR-BEC-01 : PMIOPort  Port=3  Side=Right  ConnectionType=Bus: ElectricalPower
  IF-PWR-SEC-01 : PMIOPort  Port=4  Side=Right  ConnectionType=Bus: ElectricalPower
  IF-PWR-BFC-01 : PMIOPort  Port=5  Side=Right  ConnectionType=Bus: ElectricalPower
  IF-PWR-BPR-01 : PMIOPort  Port=6  Side=Right  ConnectionType=Bus: ElectricalPower
  IF-PWR-SFC-01 : PMIOPort  Port=7  Side=Right  ConnectionType=Bus: ElectricalPower
  IF-PWR-SPR-01 : PMIOPort  Port=8  Side=Right  ConnectionType=Bus: ElectricalPower
  IF-PWR-BRA-01 : PMIOPort  Port=9  Side=Right  ConnectionType=Bus: ElectricalPower
  IF-PWR-SRA-01 : PMIOPort  Port=10  Side=Right  ConnectionType=Bus: ElectricalPower
  IF-PWR-BRX-01 : PMIOPort  Port=11  Side=Right  ConnectionType=Bus: ElectricalPower
  IF-PWR-SRX-01 : PMIOPort  Port=12  Side=Right  ConnectionType=Bus: ElectricalPower
  IF-PWR-BDX-01 : PMIOPort  Port=13  Side=Right  ConnectionType=Bus: ElectricalPower
  IF-PWR-SDX-01 : PMIOPort  Port=14  Side=Right  ConnectionType=Bus: ElectricalPower
  IF-PWR-BTA-01 : PMIOPort  Port=15  Side=Right  ConnectionType=Bus: ElectricalPower
  IF-PWR-STA-01 : PMIOPort  Port=16  Side=Right  ConnectionType=Bus: ElectricalPower
  IF-PWR-TMS-01 : PMIOPort  Port=17  Side=Right  ConnectionType=Bus: ElectricalPower
  IF-PWR-STR-01 : PMIOPort  Port=18  Side=Right  ConnectionType=Bus: ElectricalPower
  IF-PWR-GNC-01 : PMIOPort  Port=19  Side=Right  ConnectionType=Bus: ElectricalPower
  IF-PCR-HDN-01 : PMIOPort  Port=20  Side=Left  ConnectionType=Bus: ElectricalPower
  Bus Element Out3 : Outport  PortName=IF-BPI-PIS-01
  Bus Element Out2 : Outport  Port=2  PortName=IF-HSI-PIS-01
  Bus Element Out1 : Outport  Port=3  PortName=IF-HDN-PSM-01
  wires:
  Branch / Load Protection Interface/1(IF-BPI-PIS-01) -> Bus Element Out3/1
  Bus Element In1/1 -> HV Switching & Isolation/1(IF-PMC-HSI-01)
  HV Switching & Isolation/1(IF-HSI-PIS-01) -> Bus Element Out2/1
  HV Distribution Network/1(IF-HDN-PSM-01) -> Bus Element Out1/1
  connections:
  Branch / Load Protection Interface/RConn1 -- IF-PWR-GNC-01/RConn1
  Branch / Load Protection Interface/RConn7 -- IF-PWR-BDX-01/RConn1
  Branch / Load Protection Interface/RConn2 -- IF-PWR-STR-01/RConn1
  Branch / Load Protection Interface/RConn13 -- IF-PWR-SFC-01/RConn1
  Branch / Load Protection Interface/RConn6 -- IF-PWR-SDX-01/RConn1
  Branch / Load Protection Interface/RConn3 -- IF-PWR-TMS-01/RConn1
  Branch / Load Protection Interface/RConn4 -- IF-PWR-STA-01/RConn1
  Branch / Load Protection Interface/RConn5 -- IF-PWR-BTA-01/RConn1
  Branch / Load Protection Interface/RConn8 -- IF-PWR-SRX-01/RConn1
  Branch / Load Protection Interface/RConn9 -- IF-PWR-BRX-01/RConn1
  Branch / Load Protection Interface/RConn10 -- IF-PWR-SRA-01/RConn1
  Branch / Load Protection Interface/RConn11 -- IF-PWR-BRA-01/RConn1
  Branch / Load Protection Interface/RConn12 -- IF-PWR-SPR-01/RConn1
  Branch / Load Protection Interface/RConn14 -- IF-PWR-RCT-01/RConn1
  Branch / Load Protection Interface/RConn15 -- IF-PWR-TVC-01/RConn1
  Branch / Load Protection Interface/RConn16 -- IF-PWR-BEC-01/RConn1
  Branch / Load Protection Interface/RConn17 -- IF-PWR-SEC-01/RConn1
  Branch / Load Protection Interface/RConn18 -- IF-PWR-BFC-01/RConn1
  Branch / Load Protection Interface/RConn19 -- IF-PWR-BPR-01/RConn1
  IF-PCR-HDN-01/RConn1 -- HV Distribution Network/LConn1

== system StarshipSystemModel/Starship/Power & Electrical Energy/Power Conversion & Conditioning ==
  Conversion Monitoring : Subsystem
      settings: PortSchema="{\"entries\":[{\"content\":{\"headerSize\":26,\"margin\":15,\"minimumSpacing\":25,\"sides\":[{\"content\":{},\"type\":\"ConnectorPlacement.EquallySpacedRectSide\",\"uuid\":\"e231466c-79f3-4a10-9258-08b328dbb315\"},{\"content\":{\"connectorIds\":[\"Out1\"],\"side\":\"RIGHT\"},\"type\":\"ConnectorPlacement.EquallySpacedRectSide\",\"uuid\":\"d7277c0a-5b77-426a-ad5b-7f06851f857a\"},{\"content\":{\"side\":\"TOP\"},\"type\":\"ConnectorPlacement.EquallySpacedRectSide\",\"uuid\":\"72d60576-32e4-4fd9-b552-a617024da2ce\"}]},\"type\":\"ConnectorPlacement.EquallySpacedConnector\",\"uuid\":\"6309e805-37c0-4868-97b0-5f8fd0bed587\"}],\"packageUris\":[\"http://schema.mathworks.com/mf0/Connector/R2020b\"],\"version\":\"1.0\"}"
  Inverter / Conversion Function : Subsystem
      settings: PortSchema="{\"entries\":[{\"content\":{\"headerSize\":26,\"margin\":15,\"minimumSpacing\":25,\"sides\":[{\"content\":{\"connectorIds\":[\"LConn1\"]},\"type\":\"ConnectorPlacement.EquallySpacedRectSide\",\"uuid\":\"e231466c-79f3-4a10-9258-08b328dbb315\"},{\"content\":{\"connectorIds\":[\"RConn1\"],\"side\":\"RIGHT\"},\"type\":\"ConnectorPlacement.EquallySpacedRectSide\",\"uuid\":\"d7277c0a-5b77-426a-ad5b-7f06851f857a\"},{\"content\":{\"side\":\"TOP\"},\"type\":\"ConnectorPlacement.EquallySpacedRectSide\",\"uuid\":\"72d60576-32e4-4fd9-b552-a617024da2ce\"}]},\"type\":\"ConnectorPlacement.EquallySpacedConnector\",\"uuid\":\"6309e805-37c0-4868-97b0-5f8fd0bed587\"}],\"packageUris\":[\"http://schema.mathworks.com/mf0/Connector/R2020b\"],\"version\":\"1.0\"}"
  Power Conditioning / Regulation : Subsystem
      settings: PortSchema="{\"entries\":[{\"content\":{\"headerSize\":26,\"margin\":15,\"minimumSpacing\":25,\"sides\":[{\"content\":{\"connectorIds\":[\"LConn1\"]},\"type\":\"ConnectorPlacement.EquallySpacedRectSide\",\"uuid\":\"e231466c-79f3-4a10-9258-08b328dbb315\"},{\"content\":{\"connectorIds\":[\"RConn1\"],\"side\":\"RIGHT\"},\"type\":\"ConnectorPlacement.EquallySpacedRectSide\",\"uuid\":\"d7277c0a-5b77-426a-ad5b-7f06851f857a\"},{\"content\":{\"side\":\"TOP\"},\"type\":\"ConnectorPlacement.EquallySpacedRectSide\",\"uuid\":\"72d60576-32e4-4fd9-b552-a617024da2ce\"}]},\"type\":\"ConnectorPlacement.EquallySpacedConnector\",\"uuid\":\"6309e805-37c0-4868-97b0-5f8fd0bed587\"}],\"packageUris\":[\"http://schema.mathworks.com/mf0/Connector/R2020b\"],\"version\":\"1.0\"}"
  IF-BES-INV-01 : PMIOPort  Side=Left  ConnectionType=Bus: ElectricalPower
  IF-PCR-HDN-01 : PMIOPort  Port=2  Side=Right  ConnectionType=Bus: ElectricalPower
  Bus Element Out1 : Outport  PortName=IF-PCM-PSM-01
  wires:
  Conversion Monitoring/1(IF-PCM-PSM-01) -> Bus Element Out1/1
  connections:
  Power Conditioning / Regulation/RConn1 -- IF-PCR-HDN-01/RConn1
  IF-BES-INV-01/RConn1 -- Inverter / Conversion Function/LConn1
  Inverter / Conversion Function/RConn1 -- Power Conditioning / Regulation/LConn1
